simulink model "sparrow_albatros_spec_withgpio_bram"  (R2021a)
settings: Solver=VariableStepDiscrete  StartTime=0.0  StopTime=200000  RelTol=1e-3
undefined symbols (not defined in the file): pfb_coeff_gen_calc
libraries: xbsIndex_r4 x5629, casper_library_misc x33, casper_library_delays x28, xps_library x10, simulink x8, xbsReplacements_r4 x2
(part 15 of 85)

== system sparrow_albatros_spec_withgpio_bram/four_bit_quant/coeffs_pol0 ==
  addr : Inport
  data_in : Inport  Port=2
  we : Inport  Port=3
  Terminator : Terminator
  Terminator1 : Terminator
  Terminator2 : Terminator
  calc_add : Subsystem  mask{data_width=32, addr_width=11, sample_rate=sample_rate}
      mask prompts: data_width "data width"; addr_width "address width"; sample_rate "sample rate"
  convert_addr : xbsIndex_r4/Convert  gui_display_data_type=Fixed-point  arith_type=Unsigned  n_bits=addr_width  bin_pt=0  float_type=Single  exp_bits=8  fraction_bits=24  quantization=Truncate  overflow=Wrap  en=off  latency=0  pipeline=off  dbl_ovrd=off  block_type=convert
      settings: xl_area=[0, 0, 0, 0, 0, 0, 0]
  convert_din1 : xbsIndex_r4/Convert  gui_display_data_type=Fixed-point  arith_type=Unsigned  n_bits=32  bin_pt=0  float_type=Single  exp_bits=8  fraction_bits=24  quantization=Truncate  overflow=Wrap  en=off  latency=0  pipeline=off  dbl_ovrd=off  block_type=convert
      settings: xl_area=[0, 0, 0, 0, 0, 0, 0]
  convert_we : xbsIndex_r4/Convert  gui_display_data_type=Fixed-point  arith_type=Unsigned  n_bits=1  bin_pt=0  float_type=Single  exp_bits=8  fraction_bits=24  quantization=Truncate  overflow=Wrap  en=off  latency=0  pipeline=off  dbl_ovrd=off  block_type=convert
      settings: xl_area=[0, 0, 0, 0, 0, 0, 0]
  munge_in : Subsystem  AncestorBlock=casper_library_flow_control/munge  mask(munge){divisions=1, div_size=32, order=[0], arith_type_out=Unsigned, bin_pt_out=0}
      mask prompts: divisions "Number of divisions"; div_size "Division size (bits)"; order "Division packing order"; arith_type_out "Output arithmetic type"; bin_pt_out "Output binary point"
      mask help: Splits an input bus into the specified number of divisions and then recombines them in the order specified (most significant division = 0,least = number divisions-1)
      mask init:
      | munge_init(gcb, ...
      |     'divisions', divisions, ...
      |     'div_size', div_size, ...
      |     'order', order, ...
      |     'arith_type_out', arith_type_out, ...
      |     'bin_pt_out', bin_pt_out);
      settings: AttributesFormatString=|
      | split:32
      | join:0
      | Unsigned [32,0]
      mask TypeOptions arith_type_out: Unsigned | Signed  (2's comp) | Floating-point
  munge_out : Subsystem  AncestorBlock=casper_library_flow_control/munge  mask(munge){divisions=1, div_size=32, order=[0], arith_type_out=Unsigned, bin_pt_out=0}
      mask prompts: divisions "Number of divisions"; div_size "Division size (bits)"; order "Division packing order"; arith_type_out "Output arithmetic type"; bin_pt_out "Output binary point"
      mask help: Splits an input bus into the specified number of divisions and then recombines them in the order specified (most significant division = 0,least = number divisions-1)
      mask init:
      | munge_init(gcb, ...
      |     'divisions', divisions, ...
      |     'div_size', div_size, ...
      |     'order', order, ...
      |     'arith_type_out', arith_type_out, ...
      |     'bin_pt_out', bin_pt_out);
      settings: AttributesFormatString=|
      | split:32
      | join:0
      | Unsigned [32,0]
      mask TypeOptions arith_type_out: Unsigned | Signed  (2's comp) | Floating-point
  sim_mem : Subsystem  mask{arith_type=Unsigned, addr_width=11, data_width=32, data_bin_pt=0, init_vals=[2147483648  2147483648  2147483648  2147483648  2147483648  2147483648  2147483648  2147483648  2147483648  2147483648  2147483648  2147483648  2147483648  2147483648  2147483648  2147483648  2147483648  2147483648  2147483648  2147483648  2147483648  2147483648  2147483648  2147483648  2147483648  2147483648  2147483648  2147483648  2147483648  2147483648  2147483648  2147483648  2147483648  2147483648  2147483648  2147483648  2147483648  2147483648  2147483648  2147483648  2147483648  2147483648  2147483648  2147483648  2147483648  2147483648  2147483648  2147483648  2147483648  2147483648  2147483648  2147483648  2147483648  2147483648  2147483648  2147483648  2147483648  2147483648  2147483648  2147483648  2147483648  2147483648  2147483648  2147483648  2147483648  2147483648  2147483648  2147483648  2147483648  2147483648  2147483648  2147483648  2147483648  2147483648  2147483648  2147483648  2147483648  2147483648  2147483648  2147483648  2147483648  2147483648  2147483648  2147483648  2147483648  2147483648  2147483648  2147483648  2147483648  2147483648  2147483648  2147483648  2147483648  2147483648  2147483648  2147483648  2147483648  2147483648  2147483648  2147483648  2147483648  2147483648  2147483648  2147483648  2147483648  2147483648  2147483648  2147483648  2147483648  2147483648  2147483648  2147483648  2147483648  2147483648  2147483648  2147483648  2147483648  2147483648  2147483648  2147483648  2147483648  2147483648  2147483648  2147483648  2147483648  2147483648  2147483648  2147483648  2147483648  2147483648  2147483648  2147483648  2147483648  2147483648  2147483648  2147483648  2147483648  2147483648  2147483648  2147483648  2147483648  2147483648  2147483648  2147483648  2147483648  2147483648  2147483648  2147483648  2147483648  2147483648  2147483648  2147483648  2147483648  2147483648  2147483648  2147483648  2147483648  2147483648  2147483648  2147483648  2147483648  2147483648  2147483648  2147483648  2147483648  2147483648  2147483648  2147483648  2147483648  2147483648  2147483648  2147483648  2147483648  2147483648  2147483648  2147483648  2147483648  2147483648  2147483648  2147483648  2147483648  2147483648  2147483648  2147483648  2147483648  2147483648  2147483648  2147483648  2147483648  2147483648  2147483648  2147483648  2147483648  2147483648  2147483648  2147483648  2147483648  2147483648  2147483648  2147483648  2147483648  2147483648  2147483648  2147483648  2147483648  2147483648  2147483648  2147483648  2147483648  2147483648  2147483648  2147483648  2147483648  2147483648  2147483648  2147483648  2147483648  2147483648  2147483648  2147483648  2147483648  2147483648  2147483648  2147483648  2147483648  2147483648  2147483648  2147483648  2147483648  2147483648  2147483648  2147483648  2147483648  2147483648  2147483648  2147483648  2147483648  2147483648  2147483648  2147483648  2147483648  2147483648  2147483648  2147483648  2147483648  2147483648  2147483648  2147483648  2147483648  2147483648  2147483648  2147483648  2147483648  2147483648  2147483648  2147483648  2147483648  2147483648  2147483648  2147483648  2147483648  2147483648  2147483648  2147483648  2147483648  2147483648  2147483648  2147483648  2147483648  2147483648  2147483648  2147483648  2147483648  2147483648  2147483648  2147483648  2147483648  2147483648  2147483648  2147483648  2147483648  2147483648  2147483648  2147483648  2147483648  2147483648  2147483648  2147483648  2147483648  2147483648  2147483648  2147483648  2147483648  2147483648  2147483648  2147483648  2147483648  2147483648  2147483648  2147483648  2147483648  2147483648  2147483648  2147483648  2147483648  2147483648  2147483648  2147483648  2147483648  2147483648  2147483648  2147483648  2147483648  2147483648  2147483648  2147483648  2147483648  2147483648  2147483648  2147483648  2147483648  2147483648  2147483648  2147483648  2147483648  2147483648  2147483648  2147483648  2147483648  2147483648  2147483648  2147483648  2147483648 ...(+20579 chars)], sample_rate=1, csp_latency=1}
      mask prompts: arith_type "Output Data Type"; addr_width "Address width"; data_width "Data width"; data_bin_pt "Data Binary Point"; init_vals "Initial values"; sample_rate "Sample rate"; csp_latency "Latency"
      mask init:
      | % set_param([gcb, '/data_to_xilinx'], 'arith_type', arith_type)
      | % set_param([gcb, '/data_to_xilinx'], 'n_bits', get_param(gcb, 'data_width'))
      mask TypeOptions arith_type: Unsigned | Signed  (2's comp)
      mask TypeOptions data_width: 8 | 16 | 32 | 64 | 128
  sparrow_albatros_spec_withgpio_bram_four_bit_quant_coeffs_pol0_addr : xbsIndex_r4/Gateway Out  inherit_from_input=off  hdl_port=on  rows=1  columns=1  UseAsDAC=off  DACChannel='1'  interface=None  automatic_assignment=on  address_offset=hex2dec('00')  intf_name=''  intf_description=''  timing_constraint=None  locs_specified=off  LOCs={'A5','B9','A9','C1','A3','G6','E9','A6','A7','A8','B8','B1','B3','D9','B5','B4','B6','C2'}  io_standard={}  block_type=gatewayout
      settings: infoedit="Gateway out block.  Converts Xilinx fixed point inputs into ouputs of type Simulink integer, double, or fixed point.<P><P>Hardware notes:  In hardware these blocks become top level output ports or are discarded, depending on how they are configured."  sginterface={'Nallatech'=>{'xdspkit'=>{'non_memory_mapped_port'=>'uprev_Shared_BRAM_addr'}},'Xilinx'=>{'jtaghwcosim'=>{'non_memory_mapped_port'=>'uprev_Shared_BRAM_addr'},'xdspkit'=>{'non_memory_mapped_port'=>'uprev_Shared_BRAM_addr'}}}  xl_area=[0, 0, 0, 0, 0, 0, 0]
  sparrow_albatros_spec_withgpio_bram_four_bit_quant_coeffs_pol0_data_in : xbsIndex_r4/Gateway Out  inherit_from_input=off  hdl_port=on  rows=1  columns=1  UseAsDAC=off  DACChannel='1'  interface=None  automatic_assignment=on  address_offset=hex2dec('00')  intf_name=''  intf_description=''  timing_constraint=None  locs_specified=off  LOCs={'B21','B22','A22','B23','B19','C19','A20','A21','A23','B24','A24','A25','E18','D18','C18','B18'}  io_standard={}  block_type=gatewayout
      settings: infoedit="Gateway out block.  Converts Xilinx fixed point inputs into ouputs of type Simulink integer, double, or fixed point.<P><P>Hardware notes:  In hardware these blocks become top level output ports or are discarded, depending on how they are configured."  sginterface={'Nallatech'=>{'xdspkit'=>{'non_memory_mapped_port'=>'uprev_Shared_BRAM_data_in'}},'Xilinx'=>{'jtaghwcosim'=>{'non_memory_mapped_port'=>'uprev_Shared_BRAM_data_in'},'xdspkit'=>{'non_memory_mapped_port'=>'uprev_Shared_BRAM_data_in'}}}  xl_area=[0, 0, 0, 0, 0, 0, 0]
  sparrow_albatros_spec_withgpio_bram_four_bit_quant_coeffs_pol0_data_out : xbsIndex_r4/Gateway In  gui_display_data_type=Fixed-point  arith_type=Unsigned  n_bits=32  bin_pt=0  preci_type=Single  exp_width=8  frac_width=24  rows=1  columns=1  quantization=Truncate  overflow=Wrap  period=sample_rate  UseAsADC=off  ADCChannel='1'  interface=None  automatic_assignment=on  address_offset=hex2dec('00')  intf_name=''  intf_description=''  default_value=0  timing_constraint=None  locs_specified=off  LOCs={}  io_standard={}  inherit_from_input=off  hdl_port=on  dbl_ovrd=off  block_type=gatewayin
      settings: xl_area=[0, 0, 0, 0, 0, 0, 0]
  sparrow_albatros_spec_withgpio_bram_four_bit_quant_coeffs_pol0_we : xbsIndex_r4/Gateway Out  inherit_from_input=off  hdl_port=on  rows=1  columns=1  UseAsDAC=off  DACChannel='1'  interface=None  automatic_assignment=on  address_offset=hex2dec('00')  intf_name=''  intf_description=''  timing_constraint=None  locs_specified=off  LOCs={'A14'}  io_standard={}  block_type=gatewayout
      settings: infoedit="Gateway out block.  Converts Xilinx fixed point inputs into ouputs of type Simulink integer, double, or fixed point.<P><P>Hardware notes:  In hardware these blocks become top level output ports or are discarded, depending on how they are configured."  xl_area=[0, 0, 0, 0, 0, 0, 0]
  data_out : Outport  VectorParamsAs1DForOutWhenUnconnected=off
  wires:
  munge_out/1(dout) -> data_out/1
  sim_mem/1(data_out) -> sparrow_albatros_spec_withgpio_bram_four_bit_quant_coeffs_pol0_data_out/1
  sparrow_albatros_spec_withgpio_bram_four_bit_quant_coeffs_pol0_data_out/1 -> munge_out/1(din)
  convert_addr/1 -> sparrow_albatros_spec_withgpio_bram_four_bit_quant_coeffs_pol0_addr/1
  convert_din1/1 -> sparrow_albatros_spec_withgpio_bram_four_bit_quant_coeffs_pol0_data_in/1
  data_in/1 -> munge_in/1(din)
  calc_add/1(out) -> sim_mem/1(addr), convert_addr/1
  sparrow_albatros_spec_withgpio_bram_four_bit_quant_coeffs_pol0_we/1 -> Terminator2/1
  sparrow_albatros_spec_withgpio_bram_four_bit_quant_coeffs_pol0_data_in/1 -> Terminator1/1
  sparrow_albatros_spec_withgpio_bram_four_bit_quant_coeffs_pol0_addr/1 -> Terminator/1
  convert_we/1 -> sparrow_albatros_spec_withgpio_bram_four_bit_quant_coeffs_pol0_we/1
  addr/1 -> calc_add/1(in)
  we/1 -> sim_mem/3(we), convert_we/1
  munge_in/1(dout) -> sim_mem/2(data), convert_din1/1
